simulink model "serialcommunication"  (Simulink 7.4)
settings: Solver=FixedStepDiscrete  SolverMode=SingleTasking  StartTime=0.0  StopTime=inf  FixedStep=0.001  RelTol=1e-3
libraries: dsPICdrivers x5
settings Model: Creator=Danilo  LastModifiedBy=Danilo
settings OptimizationCC: OptimizeModelRefInitCode=on  LifeSpan=1
settings HardwareCC: ProdBitPerInt=16  ProdEndianess=LittleEndian  ProdWordSize=16  ProdHWDeviceType=16-bit Generic
settings RTWCC: SystemTargetFile=dspic.tlc  MakeCommand=make_CreateMPLAB  TemplateMakefile=dspic_pic30_gcc.tmf  PostCodeGenCommand=dsPIC_Compile()  Description=Embedded Target for Microchip dsPIC (real-time)  ProcessScript=dspic_make_rtw_hook
settings CodeAppCC: IgnoreCustomStorageClasses=off
settings STFCustomTargetCC: IncludeMdlTerminateFcn=off  CombineOutputUpdateFcns=on  SuppressErrorStatus=on  ERTCustomFileBanners=on  SupportContinuousTime=off  SupportNonInlinedSFcns=off  SystemTargetFile=dspic.tlc
settings ERTTargetCC: MultiwordLength=2048  ParMdlRefBuildCompliant=off  CompOptLevelCompliant=off  IncludeMdlTerminateFcn=off  SuppressErrorStatus=on  ERTFirstTimeCompliant=off  ModelStepFunctionPrototypeControlCompliant=off  CPPClassGenCompliant=off  ExtModeMexFile=ext_serial_win32_comm  InlinedParameterPlacement=NonHierarchical  ERTSrcFileBannerTemplate=dsPIC_code_template.cgt  ERTHdrFileBannerTemplate=dsPIC_code_template.cgt  ERTDataSrcFileTemplate=dsPIC_code_template.cgt  ERTDataHdrFileTemplate=dsPIC_code_template.cgt  ERTCustomFileTemplate=dsPIC_main.tlc  ConvertIfToSwitch=off
settings CustomProperty: DataType=string  Value=C:\PROGRA~2\MATLAB\R2009b\bin\win32\gmake

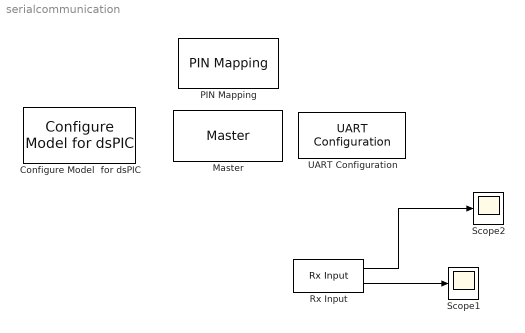
== system serialcommunication ==
  Configure Model  for dsPIC : dsPICdrivers/Simulink Configuration/Configure Model  for dsPIC
  Master : dsPICdrivers/Master  Tag=dsPIC_MASTER  Priority=1  TimeStepType=Timer1  picType=33fj64MC802  fcy=3685000  Quartz_33f=5e6  PLLActive_33f=off  fcyDesired_33f=0  tmr1="[1  3684  0]"  tmr1Info="Time Step : 0.001  ;   Error : 0%  PR1=3684"  tmr2345="[0  0  0  0]"  tmr2345cfg=[-1 -1 -1 -1]  IOautoConf=on  typePort="[ 0   0   0   0   0   0   0   0   0   0   0   0   0   0   0   0   0   0   0   0   0   0   0   0   0   0  22  23   0   0   0   0   0   0   0   0   0   0   0   0   0   0   0   0   0   0   0   0   0   0   0   0   0   0   0   0   0   0   0   0   0   0   0   0   0   0   0   0   0   0   0   0   0   0   0   0   0   0   0   0   0   0   0   0   0   0   0   0   0   0   0   0   0   0   0   0   0   0   0   0   0   0   0   0   0   0   0   0   0   0   0   0 ]"  TRIS="[ 65535  63487  65535  65535  65535  65535  65535 ]"  ADPCFG=0  MasterBusyPort=None  MasterOverloadPort=None  FOSC=Internal Fast RC 7.37Mhz  ClockSwitchMonitor=Clock switching and monitor enabled  TempProtection_33f=TEMP_ON  FPBOR=<empty>  PWRT=disable  MCLR=<empty>  ICD=ICS_PGD1  JTAGEN=JTAGEN_OFF  PowerSave=off  OverrideFcy=off  NewFcy=1e6  PR2345="[65535  65535  65535  65535]"
  PIN Mapping : dsPICdrivers/Peripheral MAPPING/PIN Mapping  Tag=dsPIC_PIN_Mapping  in_INT1=Not tied (VSS)  in_INT2=Not tied (VSS)  in_T2CK=Not tied (VSS)  in_T3CK=Not tied (VSS)  in_T4CK=Not tied (VSS)  in_T5CK=Not tied (VSS)  in_IC1=Not tied (VSS)  in_IC2=Not tied (VSS)  in_IC7=Not tied (VSS)  in_IC8=Not tied (VSS)  out_OC1=Not changed  out_OC2=Not changed  out_OC3=Not changed  out_OC4=Not changed  in_OCFA=Not tied (VSS)  in_FLTA1=Not tied (VSS)  in_FLTA2=Not tied (VSS)  in_QEA1=Not tied (VSS)  in_QEB1=Not tied (VSS)  in_INDX1=Not tied (VSS)  out_UPDN1=Not changed  out_UPDN2=Not changed  in_QEA2=Not tied (VSS)  in_QEB2=Not tied (VSS)  in_INDX2=Not tied (VSS)  in_U1RX=tied to RP10  out_U1TX=tied to RP11  in_U1CTS=Not tied (VSS)  out_U1RTS=Not changed  in_U2RX=Not tied (VSS)  out_U2TX=Not changed  in_U2CTS=Not tied (VSS)  out_U2RTS=Not changed  in_SDI1=Not tied (VSS)  out_SDO1=Not changed  in_SCK1=Not tied (VSS)  out_SCK1OUT=Not changed  in_SS1=Not tied (VSS)  out_SS1OUT=Not changed  in_SDI2=Not tied (VSS)  out_SDO2=Not changed  in_SCK2=Not tied (VSS)  out_SCK2OUT=Not changed  in_SS2=Not tied (VSS)  out_SS2OUT=Not changed  in_C1RX=Not tied (VSS)  out_C1TX=Not changed  out_C1OUT=Not changed  out_C2OUT=Not changed
  Rx Input : dsPICdrivers/Serial PORT/Rx Input  Tag=dsPIC_RX  Priority=5  UART=1  SampleTime=0.001  BlockingFctChk=on  OutputDefault=0  IsPresentFlagChk=on  OrderingInOutPopup=None
  Scope1 : Scope
      settings: YMin=-1  YMax=1
  Scope2 : Scope
      settings: YMin=-1  YMax=1
  UART Configuration : dsPICdrivers/Serial PORT/UART Configuration  Tag=dsPIC_config_UART  Priority=2  UART=1  proposed_BAUD=9600  BAUD=9600  ALT_TX_RX=off  InterruptTxWhen=When Transmit Buffer is empty  TXInterruptPri=1  TxBufferSize=32  TXEN=off  InterruptRxWhen=When Receive Buffer is full (contain 4 characters)  RXInterruptPri=7  RxBufferSize=32  DoNotImplementRxInterrupt=off  DoNotImplementTxInterrupt=off  UxBRG=23  Info="UxBRG = 23   ||  Real Baud : 9596   ||  % error : -0.037977  ||  max 0.95964 Bytes / Step"  RealBaud=0  ERROR=-0.037977  BYTES_STEP=0.95964
  wires:
  Rx Input/2 -> Scope1/1
  Rx Input/1 -> Scope2/1
